simulink model "bt_comparison_corrected"  (R2025b)
settings: Solver=ode45  StartTime=0  StopTime=30  MaxStep=0.02  RelTol=1e-8  AbsTol=1e-10
model workspace (MAT data in the model file):
  delta_u = [10; 0; 0; 0; 0]
  lin.A = [-0.35  -3.5527136788e-18; 0  0]
  lin.B = [-5e-05  0.000125  0.25  0.1  0; 0.001  0.001  0  0  -0.001]
  lin.C = [1  0; 0  1]
  lin.D = [0  0  0  0  0; 0  0  0  0  0]
  lin.fbar = [7.1054273576e-18; 0]
  lin.xbar = [0.5; 2]
  lin.ubar = [500; 200; 0.4; 0.75; 700]
  lin.is_equilibrium = 1
  lin.rho = 1000
  lin.transfer_num = {-5e-05, 0.000125, 0.25, 0.1, 0; 0.001, 0.001, 0, 0, -0.001}
  lin.transfer_den = {[1 0.35], [1 0.35], [1 0.35], [1 0.35], 1; [1 0], [1 0], 1, 1, [1 0]}
  p.rho = 1000
  p.min_volume = 1e-06
  p.Vbar = 2
  p.ubar = [500; 200; 0.4; 0.75; 700]
  p.xbar = [0.5; 2]
  p.state_names = {'solute mass fraction', 'volume'}
  p.input_names = {'w1', 'w2', 'x1', 'x2', 'wout'}
  p.input_units = {'kg/min', 'kg/min', '1', '1', 'kg/min'}
  p.state_units = {'1', 'm^3'}
  step_time = 5
  ubar = [500; 200; 0.4; 0.75; 700]
  xbar = [0.5; 2]
Description:
  | Corrected comparison at xbar=[0.5;2], ubar=[500;200;0.4;0.75;700].
  | All linear paths operate on input/state deviations; offsets are restored.
  | The transfer branch is valid for zero initial deviation only.
  | The nonlinear branch is the physical reference; linear models are local approximations.
settings Model: Creator=runner  LastModifiedBy=runner
settings DataIOCC: OutputOption=SpecifiedOutputTimes  OutputTimes=0:0.05:30

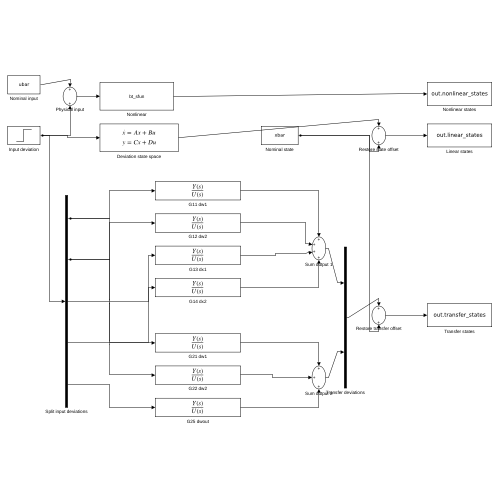
[thumbnail: Simulink's stored preview of the top-level diagram]
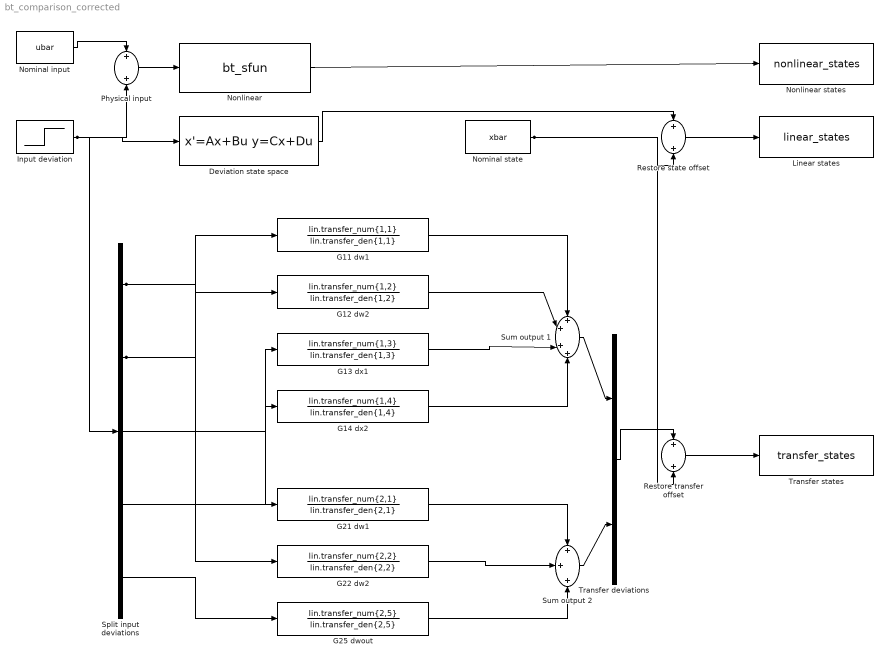
== system bt_comparison_corrected ==
  Deviation state space : StateSpace  A=lin.A  B=lin.B  C=lin.C  D=lin.D  InitialCondition=zeros(2,1)
  G11 dw1 : TransferFcn  Numerator=lin.transfer_num{1,1}  Denominator=lin.transfer_den{1,1}
  G12 dw2 : TransferFcn  Numerator=lin.transfer_num{1,2}  Denominator=lin.transfer_den{1,2}
  G13 dx1 : TransferFcn  Numerator=lin.transfer_num{1,3}  Denominator=lin.transfer_den{1,3}
  G14 dx2 : TransferFcn  Numerator=lin.transfer_num{1,4}  Denominator=lin.transfer_den{1,4}
  G21 dw1 : TransferFcn  Numerator=lin.transfer_num{2,1}  Denominator=lin.transfer_den{2,1}
  G22 dw2 : TransferFcn  Numerator=lin.transfer_num{2,2}  Denominator=lin.transfer_den{2,2}
  G25 dwout : TransferFcn  Numerator=lin.transfer_num{2,5}  Denominator=lin.transfer_den{2,5}
  Input deviation : Step  Time=step_time  Before=zeros(5,1)  After=delta_u  SampleTime=0
  Linear states : ToWorkspace  VariableName=linear_states  SaveFormat=Structure With Time  SampleTime=-1
  Nominal input : Constant  Value=ubar
  Nominal state : Constant  Value=xbar
  Nonlinear : M-S-Function  FunctionName=bt_sfun  Parameters=xbar,p
  Nonlinear states : ToWorkspace  VariableName=nonlinear_states  SaveFormat=Structure With Time  SampleTime=-1
  Physical input : Sum
  Restore state offset : Sum
  Restore transfer offset : Sum
  Split input deviations : Demux  Outputs=5
  Sum output 1 : Sum  Inputs=++++
  Sum output 2 : Sum  Inputs=+++
  Transfer deviations : Mux  Inputs=2
  Transfer states : ToWorkspace  VariableName=transfer_states  SaveFormat=Structure With Time  SampleTime=-1
  wires:
  Nominal input/1 -> Physical input/1
  Input deviation/1 -> Physical input/2, Deviation state space/1, Split input deviations/1
  Physical input/1 -> Nonlinear/1
  Nonlinear/1 -> Nonlinear states/1
  Deviation state space/1 -> Restore state offset/1
  Nominal state/1 -> Restore state offset/2, Restore transfer offset/2
  Restore state offset/1 -> Linear states/1
  Split input deviations/1 -> G11 dw1/1, G21 dw1/1
  G11 dw1/1 -> Sum output 1/1
  Split input deviations/2 -> G12 dw2/1, G22 dw2/1
  G12 dw2/1 -> Sum output 1/2
  Split input deviations/3 -> G13 dx1/1
  G13 dx1/1 -> Sum output 1/3
  Split input deviations/4 -> G14 dx2/1
  G14 dx2/1 -> Sum output 1/4
  G21 dw1/1 -> Sum output 2/1
  G22 dw2/1 -> Sum output 2/2
  Split input deviations/5 -> G25 dwout/1
  G25 dwout/1 -> Sum output 2/3
  Sum output 1/1 -> Transfer deviations/1
  Sum output 2/1 -> Transfer deviations/2
  Transfer deviations/1 -> Restore transfer offset/1
  Restore transfer offset/1 -> Transfer states/1
